simulink model "Inverter_pq_comp_sat_sim"  (R2023b)
settings: Solver=FixedStepDiscrete  StartTime=0.0  StopTime=2  RelTol=1e-3  EnableMultiTasking=on
InitFcn:
  | %% Definition of the parameters
  | 
  | Parameter_Definition
  | 
  | %% Damping
  | 
  | Rd = 3.9;
  | 
  | %% PRes Gains Calculation
  | 
  | % Definicao das grandezas
  | w_cl = 1j*2*pi*1200;  % Phase Crossing Frequency
  | no   = 1;           % Integral Resonant Constant
  | A    = 1;             % Carrier Amplitude
  | 
  | % Kp calculation
  | a0 = 1;
  | a1 = Rd*Cf;
  | b0 = 0;
  | b1 = Lf+Lg;
  | b2 = Rd*Lf*Cf+Rd*Lg*Cf;
  | b3 = Lf*Lg*Cf;
  | 
  | G_lcl = (a1*w_cl+a0)/(b3*w_cl^3+b2*w_cl^2+b1*w_cl+b0);
  | % G_lcl = 1/((Lf+Lg)*w_cl+Rf);
  | 
  | G_PWM = (1/A)*(1-w_cl*Ts/4)/(1+w_cl*Ts/4);
  | 
  | G_wc  = (Vdc/2)*(1/I_base)*G_lcl*G_PWM;
  | 
  | G_wc_abs = abs(G_wc);
  | 
  | Kp = 1/G_wc_abs;
  | 
  | % Discretized Controller Gains
  | ressonance_list = [1,5,7,11,13];
  | 
  | n_res = length(ressonance_list);
  | a = zeros(2,n_res);
  | b = zeros(2,n_res);
  | Ki_res = zeros(1,n_res);
  | 
  | % for i = 1:n_res
  | %   k = ressonance_list(i);
  | %   Ki_res(i) = (2.2*Kp)/(no*T_gr);
  | %   a(i) = (2*Ki_res(i)*Ts)/(4+((k*w_gr)^2)*Ts^2);
  | %   b(i) = (-8+2*((k*w_gr)^2)*Ts^2)/(4+((k*w_gr)^2)*Ts^2);
  | % end
  | 
  | % wc is the cutoff frequency/damping factor in rad/s
  | wc = 2;
  | 
  | for i = 1:n_res
  |   k = ressonance_list(i);
  |   wk = k * w_gr; % Resonant frequency for this harmonic
  | 
  |   Ki_res(i) = (2.2*Kp)/(0.8*no*T_gr);
  | 
  |   % 1. Calculate the common denominator
  |   den = 4 + 4*wc*Ts + (wk^2)*(Ts^2);
  | ... (+14 lines)
values from neighbouring files (symbols this model uses):
  a1_sogi = single(2*(w0_sogi^2-c_sogi^2)/den0_sogi)    [Parameter_Definition.m]
  a2_sogi = single((c_sogi^2                 - k_sogi*w0_sogi*c_sogi                 + w0_sogi^2)/den0_sogi)    [Parameter_Definition.m]
  bD_sogi = single(k_sogi*w0_sogi*c_sogi/den0_sogi)    [Parameter_Definition.m]
  bQ_sogi = single(k_sogi*w0_sogi^2/den0_sogi)    [Parameter_Definition.m]
  Cdc = 1.5e-3    (= 0.0015)    [Parameter_Definition.m]
  Cf = 5e-6    (= 5e-06)    [Parameter_Definition.m]
  f_gr = 60    [Parameter_Definition.m]
  I_base = S_base/(sqrt(3)*V_gr)    [Parameter_Definition.m]
  Lf = 1e-3    (= 0.001)    [Parameter_Definition.m]
  Lg = 0.5e-3    (= 0.0005)    [Parameter_Definition.m]
  Rdc = 0.1/(2*pi*60*Cdc)    (= 0.176838825658)    [Parameter_Definition.m]
  Rf = 0.1*Xf    (= 0.0376991118431)    [Parameter_Definition.m]
  Rg = 0.1*Xg    (= 0.0188495559215)    [Parameter_Definition.m]
  S_base = S_rated    (= 1000)    [Parameter_Definition.m]
  Ts = 2*(4167)/100e6    (= 8.334e-05)    [Parameter_Definition.m]
  Tstep = Ts/1000    (= 8.334e-08)    [Parameter_Definition.m]
  V_base = sqrt(3)*V_gr    [Parameter_Definition.m]
  V_gr = 127    [Parameter_Definition.m]
  Vdc = 800    [Parameter_Definition.m]
  Vdc_base = Vdc    (= 800)    [Parameter_Definition.m]
  w_gr = 2*pi*f_gr    (= 376.991118431)    [Parameter_Definition.m]
undefined symbols (not defined in the file or in its folder): gH_LUT, gQ_LUT, gV_LUT, lH_vetor, lQ_vetor, lV_vetor
libraries: spsSeriesRLCBranchLib x22, spsIGBTDiodeLib x12, spsCurrentMeasurementLib x9, spsVoltageMeasurementLib x5, c2837xDlib x4, spsACVoltageSourceLib x3, spsGroundLib x3, spsDCVoltageSourceLib x2, spsTriangleGeneratorLib x1, simulink x1, eeRmsMeasurement x1, spsTHDLib x1
(part 2 of 3)

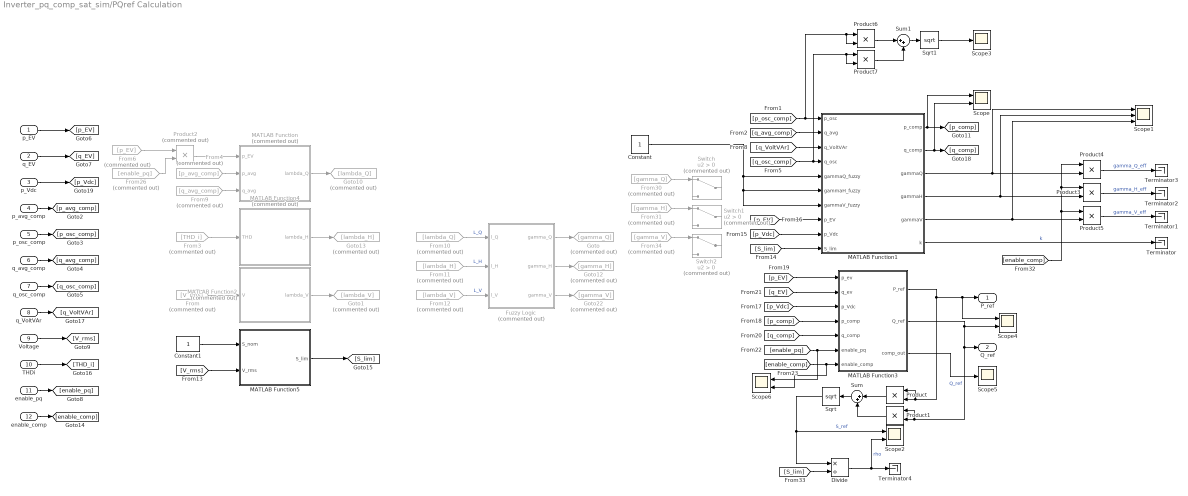
== system Inverter_pq_comp_sat_sim/PQref Calculation ==
  p_EV : Inport
  q_EV : Inport  Port=2
  p_Vdc : Inport  Port=3
  p_avg_comp : Inport  Port=4
  p_osc_comp : Inport  Port=5
  q_avg_comp : Inport  Port=6
  q_osc_comp : Inport  Port=7
  q_VoltVAr : Inport  Port=8
  Voltage : Inport  Port=9
  THDi : Inport  Port=10
  enable_pq : Inport  Port=11
  enable_comp : Inport  Port=12
  Constant : Constant  OutDataTypeStr=single  SampleTime=Ts
  Constant1 : Constant  OutDataTypeStr=single
  Divide : Product  Inputs=*/
  From : From  Commented=on  GotoTag=V_rms
  From10 : From  Commented=on  GotoTag=lambda_Q
  From11 : From  Commented=on  GotoTag=lambda_H
  From12 : From  Commented=on  GotoTag=lambda_V
  From26 : From  Commented=on  GotoTag=enable_pq
  From3 : From  Commented=on  GotoTag=THD_i
  From30 : From  Commented=on  GotoTag=gamma_Q
  From31 : From  Commented=on  GotoTag=gamma_H
  From34 : From  Commented=on  GotoTag=gamma_V
  From4 : From  Commented=on  GotoTag=p_avg_comp
  From6 : From  Commented=on  GotoTag=p_EV
  From9 : From  Commented=on  GotoTag=q_avg_comp
  Fuzzy Logic : Subsystem  Commented=on
  Goto : Goto  Commented=on  GotoTag=gamma_Q
  Goto1 : Goto  Commented=on  GotoTag=lambda_V
  Goto10 : Goto  Commented=on  GotoTag=lambda_Q
  Goto12 : Goto  Commented=on  GotoTag=gamma_H
  Goto13 : Goto  Commented=on  GotoTag=lambda_H
  Goto22 : Goto  Commented=on  GotoTag=gamma_V
  MATLAB Function : MATLAB Function  Commented=on  TreatAsAtomicUnit=on
  MATLAB Function1 : MATLAB Function  TreatAsAtomicUnit=on
  MATLAB Function2 : MATLAB Function  Commented=on  TreatAsAtomicUnit=on
  MATLAB Function3 : MATLAB Function  TreatAsAtomicUnit=on
  MATLAB Function4 : MATLAB Function  Commented=on  TreatAsAtomicUnit=on
  MATLAB Function5 : MATLAB Function  TreatAsAtomicUnit=on
  Product{,1,3..7} (7 alike) : Product
  Product2 : Product  Commented=on
  Scope{,2,4,6} (4 alike) : Scope  NumInputPorts=2
  Scope1 : Scope  NumInputPorts=3
  Scope3 : Scope
  Scope5 : Scope
  Sqrt : Sqrt
  Sqrt1 : Sqrt
  Sum : Sum  Inputs=|++
  Sum1 : Sum  Inputs=|++
  Switch : Switch  Commented=on  Criteria=u2 > Threshold  SaturateOnIntegerOverflow=off  InputSameDT=off
  Switch1 : Switch  Commented=on  Criteria=u2 > Threshold  SaturateOnIntegerOverflow=off  InputSameDT=off
  Switch2 : Switch  Commented=on  Criteria=u2 > Threshold  SaturateOnIntegerOverflow=off  InputSameDT=off
  Terminator{,1..4} (5 alike) : Terminator
  P_ref : Outport
  Q_ref : Outport  Port=2
  wires:
  Product3/1 -> Terminator2/1  "gamma_H_eff"
  From34/1 -> Switch2/1
  MATLAB Function3/1(P_ref) -> Product/2, Product/1, Scope4/1, P_ref/1
  [q_EV] -> MATLAB Function3/2(q_ev)
  Divide/1 -> Scope2/2, Terminator4/1  "rho"
  From31/1 -> Switch1/1
  Product2/1 -> MATLAB Function/1(p_EV)
  MATLAB Function1/6(k) -> Terminator/1  "k"
  Fuzzy Logic/3(gamma_V) -> Goto22/1
  Product/1 -> Sum/1
  MATLAB Function3/2(Q_ref) -> Product1/1, Product1/2, Q_ref/1, Scope4/2  "Q_ref"
  MATLAB Function1/5(gammaV) -> Scope1/3, Product5/2
  MATLAB Function1/4(gammaH) -> Scope1/2, Product3/2
  Sum/1 -> Sqrt/1
  Product5/1 -> Terminator1/1  "gamma_V_eff"
  MATLAB Function5/1(S_lim) -> [S_lim]
  [S_lim] -> Divide/2
  [enable_comp] -> Product4/1, Product3/1, Product5/1
  From9/1 -> MATLAB Function/3(q_avg)
  p_EV/1 -> [p_EV]
  p_osc_comp/1 -> [p_osc_comp]
  p_Vdc/1 -> [p_Vdc]
  Sqrt/1 -> Divide/1, Scope2/1  "S_ref"
  Constant1/1 -> MATLAB Function5/1(S_nom)
  From12/1 -> Fuzzy Logic/3(l_V)  "L_V"
  [V_rms] -> MATLAB Function5/2(V_rms)
  From10/1 -> Fuzzy Logic/1(l_Q)  "L_Q"
  [p_EV] -> MATLAB Function1/8(p_EV)
  Fuzzy Logic/2(gamma_H) -> Goto12/1
  From11/1 -> Fuzzy Logic/2(l_H)  "L_H"
  MATLAB Function1/2(q_comp) -> Scope/2, [q_comp]
  [p_osc_comp] -> MATLAB Function1/1(p_osc), Product6/2, Product6/1
  Product1/1 -> Sum/2
  [q_osc_comp] -> Product7/2, Product7/1, MATLAB Function1/4(q_osc)
  MATLAB Function1/3(gammaQ) -> Scope1/1, Product4/2
  [p_Vdc] -> MATLAB Function3/3(p_Vdc)
  Fuzzy Logic/1(gamma_Q) -> Goto/1
  q_EV/1 -> [q_EV]
  [p_Vdc] -> MATLAB Function1/9(p_Vdc)
  MATLAB Function1/1(p_comp) -> Scope/1, [p_comp]
  [S_lim] -> MATLAB Function1/10(S_lim)
  [q_VoltVAr] -> MATLAB Function1/3(q_VoltVAr)
  [p_EV] -> MATLAB Function3/1(p_ev)
  [q_comp] -> MATLAB Function3/5(q_comp)
  q_avg_comp/1 -> [q_avg_comp]
  enable_comp/1 -> [enable_comp]
  [enable_pq] -> Scope6/1, MATLAB Function3/6(enable_pq)
  From/1 -> MATLAB Function2/1(V)
  enable_pq/1 -> [enable_pq]
  MATLAB Function/1(lambda_Q) -> Goto10/1
  MATLAB Function4/1(lambda_H) -> Goto13/1
  THDi/1 -> [THD_i]
  [enable_comp] -> Scope6/2, MATLAB Function3/7(enable_comp)
  From3/1 -> MATLAB Function4/1(THD)
  [p_comp] -> MATLAB Function3/4(p_comp)
  MATLAB Function2/1(lambda_V) -> Goto1/1
  q_osc_comp/1 -> [q_osc_comp]
  Voltage/1 -> [V_rms]
  p_avg_comp/1 -> [p_avg_comp]
  q_VoltVAr/1 -> [q_VoltVAr]
  From6/1 -> Product2/1
  From4/1 -> MATLAB Function/2(p_avg)
  From30/1 -> Switch/1
  [q_avg_comp] -> MATLAB Function1/2(q_avg)
  Product4/1 -> Terminator3/1  "gamma_Q_eff"
  From26/1 -> Product2/2
  Constant/1 -> MATLAB Function1/7(gammaV_fuzzy), MATLAB Function1/6(gammaH_fuzzy), MATLAB Function1/5(gammaQ_fuzzy)
  Sum1/1 -> Sqrt1/1
  Product7/1 -> Sum1/2
  Product6/1 -> Sum1/1
  Sqrt1/1 -> Scope3/1
  MATLAB Function3/3(comp_out) -> Scope5/1

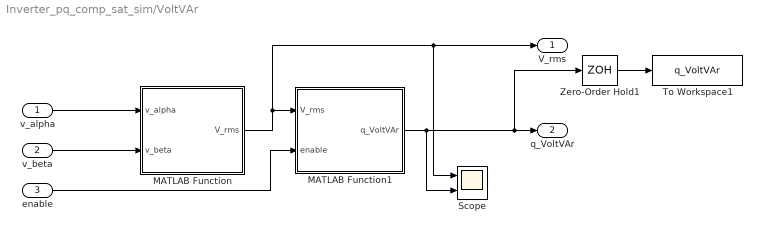
== system Inverter_pq_comp_sat_sim/VoltVAr ==
  v_alpha : Inport
  v_beta : Inport  Port=2
  enable : Inport  Port=3
  MATLAB Function : MATLAB Function  TreatAsAtomicUnit=on
  MATLAB Function1 : MATLAB Function  TreatAsAtomicUnit=on
  Scope : Scope  NumInputPorts=2
  To Workspace1 : ToWorkspace  VariableName=q_VoltVAr  SaveFormat=Timeseries  SampleTime=-1
  Zero-Order Hold1 : ZeroOrderHold  SampleTime=Ts
  V_rms : Outport
  q_VoltVAr : Outport  Port=2
  wires:
  MATLAB Function1/1(q_VoltVAr) -> Zero-Order Hold1/1, q_VoltVAr/1, Scope/2
  MATLAB Function/1(V_rms) -> Scope/1, V_rms/1, MATLAB Function1/1(V_rms)
  v_alpha/1 -> MATLAB Function/1(v_alpha)
  v_beta/1 -> MATLAB Function/2(v_beta)
  enable/1 -> MATLAB Function1/2(enable)
  Zero-Order Hold1/1 -> To Workspace1/1

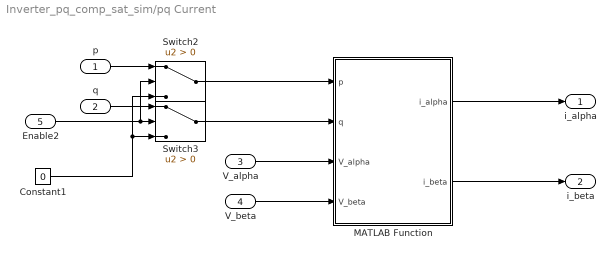
== system Inverter_pq_comp_sat_sim/pq Current ==
  p : Inport
  q : Inport  Port=2
  V_alpha : Inport  Port=3
  V_beta : Inport  Port=4
  Enable2 : Inport  Port=5
  Constant1 : Constant  Value=0
  MATLAB Function : MATLAB Function  TreatAsAtomicUnit=on
  Switch2 : Switch  Criteria=u2 > Threshold  SaturateOnIntegerOverflow=off  InputSameDT=off
  Switch3 : Switch  Criteria=u2 > Threshold  SaturateOnIntegerOverflow=off  InputSameDT=off
  i_alpha : Outport
  i_beta : Outport  Port=2
  wires:
  V_beta/1 -> MATLAB Function/4(V_beta)
  V_alpha/1 -> MATLAB Function/3(V_alpha)
  MATLAB Function/1(i_alpha) -> i_alpha/1
  MATLAB Function/2(i_beta) -> i_beta/1
  p/1 -> Switch2/1
  Switch3/1 -> MATLAB Function/2(q)
  q/1 -> Switch3/1
  Constant1/1 -> Switch2/3, Switch3/3
  Enable2/1 -> Switch2/2, Switch3/2
  Switch2/1 -> MATLAB Function/1(p)

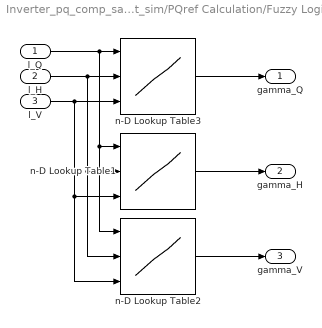
== system Inverter_pq_comp_sat_sim/PQref Calculation/Fuzzy Logic ==
  l_Q : Inport
  l_H : Inport  Port=2
  l_V : Inport  Port=3
  n-D Lookup Table1 : Lookup_n-D  NumberOfTableDimensions=3  BreakpointsForDimension1=lQ_vetor  BreakpointsForDimension2=lH_vetor  BreakpointsForDimension3=lV_vetor  Table=gH_LUT  InternalRulePriority=Speed  RndMeth=Simplest
      settings: InputPortMap=u0,u1,u2
  n-D Lookup Table2 : Lookup_n-D  NumberOfTableDimensions=3  BreakpointsForDimension1=lQ_vetor  BreakpointsForDimension2=lH_vetor  BreakpointsForDimension3=lV_vetor  Table=gV_LUT  InternalRulePriority=Speed  RndMeth=Simplest
      settings: InputPortMap=u0,u1,u2
  n-D Lookup Table3 : Lookup_n-D  NumberOfTableDimensions=3  BreakpointsForDimension1=lQ_vetor  BreakpointsForDimension2=lH_vetor  BreakpointsForDimension3=lV_vetor  Table=gQ_LUT  InternalRulePriority=Speed  RndMeth=Simplest
      settings: InputPortMap=u0,u1,u2
  gamma_Q : Outport
  gamma_H : Outport  Port=2
  gamma_V : Outport  Port=3
  wires:
  l_V/1 -> n-D Lookup Table3/3, n-D Lookup Table2/3, n-D Lookup Table1/3
  l_Q/1 -> n-D Lookup Table3/1, n-D Lookup Table2/1, n-D Lookup Table1/1
  l_H/1 -> n-D Lookup Table3/2, n-D Lookup Table2/2, n-D Lookup Table1/2
  n-D Lookup Table3/1 -> gamma_Q/1
  n-D Lookup Table1/1 -> gamma_H/1
  n-D Lookup Table2/1 -> gamma_V/1

== matlab function Inverter_pq_comp_sat_sim/RMS_fcn4 ==
  data: RMSin input; yout output
function yout = fcn(RMSin)

win = 200;

persistent sampleRMS
    if isempty(sampleRMS)
        sampleRMS = single(0.0);
    end
    if sampleRMS>=win
        sampleRMS = single(0.0);
    end

persistent RMSout
if isempty(RMSout)
    RMSout = single(0.0);
end    
persistent sumRMS
if isempty(sumRMS)
    sumRMS = single(0.0);
end
persistent RMSinArray
     if isempty(RMSinArray)
         RMSinArray = zeros(1,win);
     end

sampleRMS = sampleRMS + 1;      

%RMS of Input Signal
sumRMS = sumRMS + RMSin*RMSin - RMSinArray(1,sampleRMS);
RMSinArray(1,sampleRMS) = RMSin*RMSin;
if sumRMS>=0.0
    RMSout = sqrt(sumRMS/win);
end

%RMSout = RMSout_temp;

yout = RMSout;

== matlab function Inverter_pq_comp_sat_sim/RMS_fcn5 ==
  data: RMSin input; yout output
function yout = fcn(RMSin)

win = 200;

persistent sampleRMS
    if isempty(sampleRMS)
        sampleRMS = single(0.0);
    end
    if sampleRMS>=win
        sampleRMS = single(0.0);
    end

persistent RMSout
if isempty(RMSout)
    RMSout = single(0.0);
end    
persistent sumRMS
if isempty(sumRMS)
    sumRMS = single(0.0);
end
persistent RMSinArray
     if isempty(RMSinArray)
         RMSinArray = zeros(1,win);
     end

sampleRMS = sampleRMS + 1;      

%RMS of Input Signal
sumRMS = sumRMS + RMSin*RMSin - RMSinArray(1,sampleRMS);
RMSinArray(1,sampleRMS) = RMSin*RMSin;
if sumRMS>=0.0
    RMSout = sqrt(sumRMS/win);
end

%RMSout = RMSout_temp;

yout = RMSout;

== matlab function Inverter_pq_comp_sat_sim/Compensation Reference/MATLAB Function1 ==
  data: i_alpha input; p_avg output; i_beta input; v_alpha input; v_beta input; p_osc output; q_avg output; q_osc output
function [p_avg, p_osc, q_avg, q_osc] = pqCalc(i_alpha, i_beta, v_alpha, v_beta)
    % Initial logic and parameters are validated. 
    % Standard processing applied for spatial vector alignment.

    persistent buffer_p buffer_q sum_p sum_q idx
    window = 200; % Must match your 12000Hz/60Hz window size exactly
    
    if isempty(buffer_p)
        buffer_p = zeros(window, 1);
        buffer_q = zeros(window, 1);
        sum_p = single(0.0);
        sum_q = single(0.0);
        idx = 1;
    end
    
    % Final transformation: Strip scaling coefficients to match I_total_sq domain
    p = (v_alpha * i_alpha) + (v_beta * i_beta);
    q = (v_beta * i_alpha) - (v_alpha * i_beta);
    
    % Align filter topology to match current/voltage sliding window
    old_p = buffer_p(idx);
    old_q = buffer_q(idx);
    
    buffer_p(idx) = p;
    buffer_q(idx) = q;
    
    sum_p = sum_p + p - old_p;
    sum_q = sum_q + q - old_q;
    
    idx = idx + 1;
    if idx > window
        idx = 1;
    end
    
    p_avg = sum_p / window;
    q_avg = sum_q / window;
    
    p_osc = p - p_avg;
    q_osc = q - q_avg;
end

== matlab function Inverter_pq_comp_sat_sim/MATLAB Function11 ==
  data: i_rms input; error_overcurrent output; error_ac_overvoltage output; error_dc_overvoltage output; error_unbalance output; error_low_Vdc output; enable_contactor_out output; enable_PreCharge_out output; enable_PWM_out output; enable_PQ_out output; enable_comp_out output; enable_Feedforward_out output; I_limit input; V_rms input; V_limit input; V_dc input; Vdc_limit input; V_unb input; Vunb_limit input; enable_relay input; enable_PWM input; enable_PreCharge input; enable_PQ input; enable_comp input; error_reset input; error_reset_out output; out_gpio output
function [error_overcurrent, error_ac_overvoltage, error_dc_overvoltage, error_unbalance, error_low_Vdc, enable_contactor_out, enable_PreCharge_out, enable_PWM_out, enable_PQ_out, enable_comp_out, enable_Feedforward_out, error_reset_out, out_gpio] = TNPC_Protection(i_rms, I_limit, V_rms, V_limit, V_dc, Vdc_limit, V_unb, Vunb_limit, enable_relay, enable_PWM, enable_PreCharge, enable_PQ, enable_comp, error_reset)

% Persistent variables definition
persistent error_flag
persistent error_overcurrent_p
persistent error_ac_overvoltage_p
persistent error_dc_overvoltage_p
persistent error_unbalance_p
persistent error_low_Vdc_p
persistent count_I_limit
if isempty(error_flag)
    error_flag = single(0);
    error_overcurrent_p    = single(0);
    error_ac_overvoltage_p = single(0);
    error_dc_overvoltage_p = single(0);
    error_unbalance_p      = single(0);
    error_low_Vdc_p        = single(0);
    count_I_limit          = int16(0);
end


out_Feedforward = single(0.0);
% Count to keep high current limit in first 15 cycles
if enable_relay == 1
    if count_I_limit < 10*200
        I_limit = single(100.0);
        count_I_limit = count_I_limit + 1;
        out_Feedforward = single(1.0);
    elseif count_I_limit < 15*200
        I_limit = single(100.0);
        count_I_limit = count_I_limit + 1;
        out_Feedforward = single(0.0);
    end
end

enable_Feedforward_out = out_Feedforward;

% Check for errors
if max(i_rms) > I_limit
    error_overcurrent = single(1);
    error_overcurrent_p = single(1);
else
    error_overcurrent = single(0);
end

if V_dc > Vdc_limit
    error_dc_overvoltage = single(1);
    error_dc_overvoltage_p = single(1);
else
    error_dc_overvoltage = single(0);  
end

if V_unb > Vunb_limit
    error_unbalance = single(1);
    error_unbalance_p = single(1);
else
    error_unbalance = single(0);
end

if max(V_rms) > V_limit
    error_ac_overvoltage = single(1);
    error_ac_overvoltage_p = single(1);
else
    error_ac_overvoltage = single(0);  
end

if V_dc*500 < sqrt(2)*max(V_rms)*250
    error_low_Vdc = single(1);
    error_low_Vdc_p = single(1);
else
    error_low_Vdc = single(0);
end

% Raise the error flag
if (error_overcurrent == 1) || (error_dc_overvoltage == 1) || (error_unbalance == 1) || (error_ac_overvoltage == 1) || (error_low_Vdc == 1)
    error_flag = single(1);
end

% Reset logic
if error_flag == 1 && error_reset == 1 && error_overcurrent == 0 && error_dc_overvoltage == 0 && error_ac_overvoltage == 0 && error_unbalance == 0 && error_low_Vdc == 0
    % Clear the persistent variables
    error_flag = single(0);
    error_overcurrent_p    = single(0);
    error_ac_overvoltage_p = single(0);
    error_dc_overvoltage_p = single(0);
    error_unbalance_p      = single(0);
    error_low_Vdc_p        = single(0);
    count_I_limit          = int16(0);
    % Send 0 to the reset signal
    error_reset_out = single(0);
else
    error_reset_out = error_reset;
end

% Enable signals output
if error_flag == 1
    enable_contactor_out = single(0);
    enable_PWM_out       = single(0);
    enable_PreCharge_out = single(0);
    enable_PQ_out        = single(0);
    enable_comp_out      = single(0);
else
    enable_contactor_out = enable_relay;
    enable_PWM_out       = enable_PWM;
    enable_PreCharge_out = enable_PreCharge;
    enable_PQ_out        = enable_PQ;
    enable_comp_out      = enable_comp;
end

if (error_overcurrent_p == 1) || (error_dc_overvoltage_p == 1) || (error_unbalance_p == 1) || (error_ac_overvoltage_p == 1) || (error_low_Vdc_p == 1)
    out_gpio = single(1);
else
    out_gpio = single(0);
end

== matlab function Inverter_pq_comp_sat_sim/PQref Calculation/MATLAB Function ==
  data: p_EV input; p_avg input; lambda_Q output; q_avg input
function lambda_Q  = lambda_Q_calc(p_EV, p_avg, q_avg)

lQ_min = sqrt(1-0.75^2);

lQ = q_avg/sqrt((-p_EV + p_avg)^2+q_avg^2);
lambda_Q = lQ/lQ_min;
lambda_Q = max(-1,min(1,lambda_Q));

== matlab function Inverter_pq_comp_sat_sim/Current Controller/RMS_fcn ==
  data: RMSin input; yout output
function yout = fcn(RMSin)

win = 200;

persistent sampleRMS
    if isempty(sampleRMS)
        sampleRMS = single(0.0);
    end
    if sampleRMS>=win
        sampleRMS = single(0.0);
    end

persistent RMSout
if isempty(RMSout)
    RMSout = single(0.0);
end    
persistent sumRMS
if isempty(sumRMS)
    sumRMS = single(0.0);
end
persistent RMSinArray
     if isempty(RMSinArray)
         RMSinArray = zeros(1,win);
     end

sampleRMS = sampleRMS + 1;      

%RMS of Input Signal
sumRMS = sumRMS + RMSin*RMSin - RMSinArray(1,sampleRMS);
RMSinArray(1,sampleRMS) = RMSin*RMSin;
if sumRMS>=0.0
    RMSout = sqrt(sumRMS/win);
end

%RMSout = RMSout_temp;

yout = RMSout;

== matlab function Inverter_pq_comp_sat_sim/PQref Calculation/MATLAB Function1 ==
  data: p_osc input; q_avg input; q_VoltVAr input; q_osc input; gammaQ_fuzzy input; gammaH_fuzzy input; gammaV_fuzzy input; p_comp output; q_comp output; p_EV input; p_Vdc input; S_lim input; gammaQ output; gammaH output; gammaV output; k output
function [p_comp, q_comp, gammaQ, gammaH, gammaV, k] = PQCompCalc( ...
    p_osc, q_avg, q_VoltVAr, q_osc, ...
    gammaQ_fuzzy, gammaH_fuzzy, gammaV_fuzzy, p_EV, p_Vdc, S_lim)
%#codegen

    window = 200;
    eps_power = single(1e-9);

    % Monotonic maximum deque for S_total
    persistent q_Stotal;
    persistent pos_Stotal;

    % Monotonic minimum deque for k
    persistent q_k;
    persistent pos_k;

    persistent t;

    if isempty(t)
        q_Stotal = zeros(window, 2, "single");
        q_k      = zeros(window, 2, "single");

        pos_Stotal = 0;
        pos_k = 0;
        t = 0;
    end

    % ---------------------------------------------------------------------
    % Sample counter
    % ---------------------------------------------------------------------
    t = t + 1;

    if t > 1000000
        for i = 1:pos_Stotal
            q_Stotal(i, 2) = q_Stotal(i, 2) - 1000000;
        end

        for i = 1:pos_k
            q_k(i, 2) = q_k(i, 2) - 1000000;
        end

        t = t - 1000000;
    end

    % Maintain your adopted p_Vdc sign convention.
    p_0 = p_EV - p_Vdc;

    % Ensure a nonnegative limit
    S_lim_safe = max(S_lim, single(0.0));

    % =====================================================================
    % 1. ROLLING MAXIMUM OF THE TOTAL REQUIRED POWER
    % =====================================================================
    S_tot_inst = sqrt( ...
        (p_0 + p_osc)^2 + ...
        (q_avg + q_VoltVAr + q_osc)^2);

    % ---------------------------------------------------------------------
    % IMPORTANT CORRECTION:
    % Remove expired samples BEFORE inserting the new sample.
    % ---------------------------------------------------------------------
    while (pos_Stotal > 0) && ...
          (q_Stotal(1, 2) <= t - window)

        for i = 1:(pos_Stotal - 1)
            q_Stotal(i, :) = q_Stotal(i + 1, :);
        end

        pos_Stotal = pos_Stotal - 1;
    end

    % Remove samples dominated by the current value
    while (pos_Stotal > 0) && ...
          (q_Stotal(pos_Stotal, 1) <= S_tot_inst)

        pos_Stotal = pos_Stotal - 1;
    end

    % Defensive protection. With the expiration order corrected,
    % this condition should normally never occur.
    if pos_Stotal >= window
        for i = 1:(window - 1)
            q_Stotal(i, :) = q_Stotal(i + 1, :);
        end

        pos_Stotal = window - 1;
    end

    % Insert current sample
    pos_Stotal = pos_Stotal + 1;
    q_Stotal(pos_Stotal, 1) = S_tot_inst;
    q_Stotal(pos_Stotal, 2) = t;

    % Maximum is always stored at the beginning of the deque
    S_total_max = q_Stotal(1, 1);

    % =====================================================================
    % 2. FUZZY-WEIGHTED COMPENSATION REFERENCES
    % =====================================================================
    p_fuz = gammaH_fuzzy * p_osc;

    q_fuz = gammaQ_fuzzy * q_avg + gammaV_fuzzy * q_VoltVAr + gammaH_fuzzy  * q_osc;

    % Maximum scaling allowed without overcompensation
    lambda_max = max(gammaV_fuzzy, max(gammaQ_fuzzy, gammaH_fuzzy));

    if lambda_max > eps_power
        k_cap = single(1.0) / lambda_max;
    else
        % Both fuzzy weights are zero. The value of k has no effect
        % because p_fuz = q_fuz = 0.
        k_cap = single(1.0);
    end

    % Quadratic coefficients
    a = p_fuz^2 + q_fuz^2;
    b = 2 * p_0 * p_fuz;
    c = p_0^2 - S_lim_safe^2;

    % Indicates whether a meaningful k value exists at this sample
    update_k_queue = true;

    if a < eps_power
        % No ancillary-service vector exists at this instant.
        %
        % Do not use k_inst = 0, because it would remain in the minimum
        % queue for one complete grid cycle and temporarily block
        % compensation when a load is connected.
        k_inst = k_cap;
        update_k_queue = false;

    else
        delta = b^2 - 4 * a * c;

        if delta < 0
            % A slightly negative value can be caused by rounding.
            % A significantly negative value normally indicates that
            % the requested operating point is infeasible.
            delta = single(0.0);
        end

        % Largest root: maximum positive scaling that satisfies S_lim
        k_inst = (-b + sqrt(delta)) / (2 * a);

        % Prevent negative scaling and overcompensation
        k_inst = max(k_inst, single(0.0));
        k_inst = min(k_inst, k_cap);
    end

    % =====================================================================
    % 3. ROLLING MINIMUM OF k
    % =====================================================================

    % Remove all expired k samples before inserting a new one
    while (pos_k > 0) && (q_k(1, 2) <= t - window)

        for i = 1:(pos_k - 1)
            q_k(i, :) = q_k(i + 1, :);
        end

        pos_k = pos_k - 1;
    end

    % Only store k when the compensation vector is meaningful
    if update_k_queue

        % Remove values dominated by the current minimum candidate
        while (pos_k > 0) && ...
              (q_k(pos_k, 1) >= k_inst)

            pos_k = pos_k - 1;
        end

        % Defensive overflow protection
        if pos_k >= window
            for i = 1:(window - 1)
                q_k(i, :) = q_k(i + 1, :);
            end

            pos_k = window - 1;
        end

        % Insert current k
        pos_k = pos_k + 1;
        q_k(pos_k, 1) = k_inst;
        q_k(pos_k, 2) = t;
    end

    % Obtain the rolling minimum
    if pos_k > 0
        k_min = q_k(1, 1);
    else
        % No valid compensation demand has been observed
        k_min = k_cap;
    end

    % Apply current-sample protection again because the fuzzy
    % weights, and therefore k_cap, may have changed.
    k_min = max(k_min, single(0.0));
    k_min = min(k_min, k_cap);

    % =====================================================================
    % 4. FINAL COMPENSATION REFERENCES
    % =====================================================================
    if S_total_max <= S_lim_safe

        % Full compensation is feasible
        p_comp = p_osc;
        q_comp = q_avg + q_VoltVAr + q_osc;

        gammaQ = single(1.0);
        gammaH = single(1.0);
        gammaV = single(1.0);
        k = single(1.0);

    else

        % Insufficient converter capacity
        p_comp = k_min * p_fuz;
        q_comp = k_min * q_fuz;

        gammaQ = min(gammaQ_fuzzy * k_min, 1);
        gammaH  = min(gammaH_fuzzy  * k_min, 1);
        gammaV  = min(gammaV_fuzzy  * k_min, 1);
        k = k_min;
    end
end

== matlab function Inverter_pq_comp_sat_sim/MATLAB Function6 ==
  data: i_alpha input; p_avg output; i_beta input; v_alpha input; v_beta input; p_osc output; q_avg output; q_osc output
function [p_avg, p_osc, q_avg, q_osc] = pqCalc(i_alpha, i_beta, v_alpha, v_beta)
    % Initial logic and parameters are validated. 
    % Standard processing applied for spatial vector alignment.

    persistent buffer_p buffer_q sum_p sum_q idx
    window = 200; % Must match your 12000Hz/60Hz window size exactly
    
    if isempty(buffer_p)
        buffer_p = zeros(window, 1, "single");
        buffer_q = zeros(window, 1, "single");
        sum_p = single(0.0);
        sum_q = single(0.0);
        idx = 1;
    end
    
    % Final transformation: Strip scaling coefficients to match I_total_sq domain
    p = (v_alpha * i_alpha) + (v_beta * i_beta);
    q = (v_beta * i_alpha) - (v_alpha * i_beta);
    
    % Align filter topology to match current/voltage sliding window
    old_p = buffer_p(idx);
    old_q = buffer_q(idx);
    
    buffer_p(idx) = p;
    buffer_q(idx) = q;
    
    sum_p = sum_p + p - old_p;
    sum_q = sum_q + q - old_q;
    
    idx = idx + 1;
    if idx > window
        idx = 1;
    end
    
    p_avg = sum_p / window;
    q_avg = sum_q / window;
    
    p_osc = p - p_avg;
    q_osc = q - q_avg;
end

== matlab function Inverter_pq_comp_sat_sim/Current Controller/MATLAB Function2 ==
  data: alpha input; a output; beta input; b output; c output; aux output
function [a, b, c, aux] = abc(alpha, beta)

a = sqrt(2/3)*alpha;
b = sqrt(2/3)*(-1*alpha/2 + sqrt(3)*beta/2);
c = sqrt(2/3)*(-1*alpha/2 - sqrt(3)*beta/2);

max_mod = max(abs([a, b, c]));

if max_mod > 1
    % scale = 1/max_mod;
    % 
    % a = a*scale;
    % b = b*scale;
    % c = c*scale;

    aux = single(1.0);
else
    aux = single(0.0);
end

== matlab function Inverter_pq_comp_sat_sim/PQref Calculation/MATLAB Function2 ==
  data: V input; lambda_V output
function lambda_V = lambda_V_calc(V)

delta_V = 0.15;
V_min = 1-delta_V;
V_max = 1+delta_V;

lambda_V = (V-V_min)/(V_max-V_min);
lambda_V = max(0,min(1,lambda_V));

== matlab function Inverter_pq_comp_sat_sim/MATLAB Function3 ==
  data: a input; alpha output; b input; c input; beta output
function [alpha, beta] = alpha_beta(a, b, c)

alpha = sqrt(2/3)*(a - b/2 - c/2);
beta  = sqrt(2/3)*(sqrt(3)*b/2 - sqrt(3)*c/2);

== matlab function Inverter_pq_comp_sat_sim/pq Current/MATLAB Function ==
  data: p input; i_alpha output; q input; i_beta output; V_alpha input; V_beta input
function [i_alpha, i_beta] = pq_to_i(p, q, V_alpha, V_beta)

i_alpha = (1/(V_alpha^2+V_beta^2))*(V_alpha*p + V_beta*q);
i_beta  = (1/(V_alpha^2+V_beta^2))*(V_beta*p - V_alpha*q);

== matlab function Inverter_pq_comp_sat_sim/PQref Calculation/MATLAB Function3 ==
  data: p_ev input; P_ref output; q_ev input; p_Vdc input; p_comp input; q_comp input; enable_pq input; enable_comp input; Q_ref output; comp_out output
function [P_ref, Q_ref,comp_out] = PQ_ref(p_ev, q_ev, p_Vdc, p_comp, q_comp, enable_pq, enable_comp)

comp_out = 0;
if enable_pq == 0
    P_ref = -1*p_Vdc;
    Q_ref = single(0.0);
else
    if enable_comp == 0
        P_ref = p_ev - p_Vdc;
        Q_ref = q_ev;
    else
        P_ref = p_ev - p_Vdc + p_comp;
        Q_ref = q_ev + q_comp;
        comp_out = 1;
    end
end

== matlab function Inverter_pq_comp_sat_sim/PQref Calculation/MATLAB Function4 ==
  data: THD input; lambda_H output
function lambda_H  = lambda_H_calc(THD)

THD_min = 0;
THD_max = 0.3;

% Number of samples in the MAF window
% Set this equal to approximately one grid cycle
N_MAF = 200;

% ---------------------------------------------------------
% Moving Average Filter
% ---------------------------------------------------------
persistent buffer idx count running_sum

if isempty(buffer)
    buffer = zeros(1, N_MAF);
    idx = 1;
    count = 0;
    running_sum = 0;
end

% Remove oldest value from running sum
running_sum = running_sum - buffer(idx);

% Store new value
buffer(idx) = THD;

% Add new value to running sum
running_sum = running_sum + THD;

% Number of valid samples during startup
if count < N_MAF
    count = count + 1;
end

% Calculate moving average
THD = running_sum / count;

% Advance circular-buffer index
idx = idx + 1;

if idx > N_MAF
    idx = 1;
end

lambda_H = (THD - THD_min)/(THD_max - THD_min);
% Saturation [0,1]
lambda_H = max(0, min(1, lambda_H));

== matlab function Inverter_pq_comp_sat_sim/Compensation Reference/MATLAB Function ==
  data: i_alpha input; THDi output; i_beta input; v_alpha input; v_beta input; p_EV input; p_avg input; q_avg input
function THDi = THD_calc( ...
    i_alpha, i_beta, ...
    v_alpha, v_beta, ...
    p_EV, p_avg, q_avg)
%#codegen

    window = 200;
    epsilon = 1e-9;

    persistent buffer_I_total;
    persistent buffer_V;
    persistent sum_I_total;
    persistent sum_V;
    persistent idx;
    persistent count;

    if isempty(idx)
        buffer_I_total = zeros(window,1);
        buffer_V = zeros(window,1);

        sum_I_total = single(0.0);
        sum_V = single(0.0);

        idx = 1;
        count = 0;
    end

    % Load-current magnitude squared
    I_total_inst_sq = i_alpha^2 + i_beta^2;

    % Fundamental PCC-voltage magnitude squared
    V_inst_sq = v_alpha^2 + v_beta^2;

    % Remove oldest samples
    old_I = buffer_I_total(idx);
    old_V = buffer_V(idx);

    % Insert newest samples
    buffer_I_total(idx) = I_total_inst_sq;
    buffer_V(idx) = V_inst_sq;

    % Update moving sums
    sum_I_total = ...
        sum_I_total + I_total_inst_sq - old_I;

    sum_V = ...
        sum_V + V_inst_sq - old_V;

    idx = idx + 1;

    if idx > window
        idx = 1;
    end

    if count < window
        count = count + 1;
    end

    % Do not calculate THD before one complete cycle
    if count < window
        THDi = single(0.0);
        return;
    end

    % Squared total load-current magnitude
    IL_total_sq = max(sum_I_total/window,single(0.0));

    % Squared fundamental voltage magnitude
    V1_sq = max(sum_V/window,epsilon);

    % Fundamental LOAD current
    IL_fund_sq = ...
        (p_avg^2 + q_avg^2)/V1_sq;

    % Harmonic LOAD current
    IH_load_sq = max( ...
        IL_total_sq - IL_fund_sq, ...
        single(0.0));

    % Fundamental grid current including EV charging
    %
    % Current convention:
    % p_EV is negative during charging.
    p_total_fund = p_avg - p_EV;

    IT_fund_sq = ...
        (p_total_fund^2 + q_avg^2)/V1_sq;

    % Equivalent pre-compensation grid THD
    if IT_fund_sq <= epsilon
        THDi = single(0.0);
    else
        THDi = sqrt(IH_load_sq/IT_fund_sq);
    end
end

== matlab function Inverter_pq_comp_sat_sim/VoltVAr/MATLAB Function ==
  data: v_alpha input; V_rms output; v_beta input
function V_rms = VrmsCalc(v_alpha, v_beta)
    % #codegen
    window = 200;
    
    
    persistent buffer;
    persistent idx;
    persistent sum_vsq;
    
    % Inicialização
    if isempty(idx)
        buffer = zeros(window, 1);
        idx = 1;
        sum_vsq = single(0.0);
    end
    
    % 1. Calcula o quadrado da magnitude instantânea (V_alpha^2 + V_beta^2)
    v_sq_inst = v_alpha^2 + v_beta^2;
    
    % 2. Média Móvel Rápida (Soma o novo, subtrai o mais antigo do buffer)
    sum_vsq = sum_vsq - buffer(idx) + v_sq_inst;
    
    % Atualiza a memória com o novo valor
    buffer(idx) = v_sq_inst;
    
    % Avança o ponteiro circular
    idx = idx + 1;
    if idx > window
        idx = 1;
    end
    
    % 3. Calcula a média e extrai a raiz para obter o RMS
    % Garante que a soma não seja negativa por erro de precisão flutuante (max)
    v_sq_medio = max(sum_vsq / window, 0);
    
    % Equação final: V_rms = V_pico / sqrt(2) = sqrt(V_sq_medio / 2)
    V_rms = sqrt(v_sq_medio);
    
end

== matlab function Inverter_pq_comp_sat_sim/VoltVAr/MATLAB Function1 ==
  data: V_rms input; q_VoltVAr output; enable input
function q_VoltVAr = VoltVAr(V_rms, enable)

% Curve Definition
V1 = 0.9;
V2 = 0.96;
V3 = 1.03;
V4 = 1.10;

% Max Q processing
Q_max = single(1.0);

if enable == 0
    q_VoltVAr = single(0.0);
else
    if V_rms < V1
        q_VoltVAr = Q_max;
    else
        if V_rms < V2
            q_VoltVAr = Q_max*(V2 - V_rms)/(V2 - V1);
        else
            if V_rms < V3
                q_VoltVAr = single(0.0);
            else
               if V_rms < V4
                   q_VoltVAr = single(-1.0)*Q_max*(V_rms - V3)/(V4 - V3);
               else
                   q_VoltVAr = single(-1.0)*Q_max;
               end
            end
        end
    end
end

== matlab function Inverter_pq_comp_sat_sim/MATLAB Function5 ==
  data: a input; alpha output; b input; c input; beta output
function [alpha, beta] = alpha_beta(a, b, c)

alpha = sqrt(2/3)*(a - b/2 - c/2);
beta  = sqrt(2/3)*(sqrt(3)*b/2 - sqrt(3)*c/2);

== matlab function Inverter_pq_comp_sat_sim/Current Controller/PRes ==
  data: Kp input; a input; b input; errora input; ma output; errorb input; mb output; enable input
function [ma, mb] = PResCurrent(Kp, a, b, errora, errorb, enable)

%Controller modeled in abc frame, considering p.u. values

%%% Variables Definition
%%%%#########################################################
%%%%######################################################### 

nRes = length(a);

max_pu = single(1.0);

%Proportional part variable
%Phase a
persistent pia
    if isempty(pia)
        pia = single(0.0);
    end
%Phase b    
persistent pib
    if isempty(pib)
        pib = single(0.0);
    end 
    
%Resonant parts variables
%Phase a
persistent presa
    if isempty(presa)
        presa = zeros(1,nRes);
    end
persistent presa_1d %1 sample delay
    if isempty(presa_1d)
        presa_1d = zeros(1,nRes);
    end    
persistent presa_2d %2 samples delay
    if isempty(presa_2d)
        presa_2d = zeros(1,nRes);
    end
persistent presOUT_ia
    if isempty(presOUT_ia)
        presOUT_ia = single(0.0);
    end
    
%Phase b
persistent presb
    if isempty(presb)
        presb = zeros(1,nRes);
    end
persistent presb_1d %1 sample delay
    if isempty(presb_1d)
        presb_1d = zeros(1,nRes);
    end    
persistent presb_2d %2 samples delay
    if isempty(presb_2d)
        presb_2d = zeros(1,nRes);
    end
persistent presOUT_ib
    if isempty(presOUT_ib)
        presOUT_ib = single(0.0);
    end

%Error variables
%Phase a
% persistent errora %Actual error
%     if isempty(errora)
%         errora = 0.0;
%     end
persistent errora_0d %Actual error to delay
    if isempty(errora_0d)
        errora_0d = single(0.0);
    end
persistent errora_1d %1 sample delay
    if isempty(errora_1d)
        errora_1d = single(0.0);
    end    
persistent errora_2d %2 sample delay
    if isempty(errora_2d)
        errora_2d = single(0.0);
    end   
%Phase b
% persistent errorb %Actual error
%     if isempty(errorb)
%         errorb = 0.0;
%     end
persistent errorb_0d %Actual error to delay
    if isempty(errorb_0d)
        errorb_0d = single(0.0);
    end
persistent errorb_1d %1 sample delay
    if isempty(errorb_1d)
        errorb_1d = single(0.0);
    end    
persistent errorb_2d %2 sample delay
    if isempty(errorb_2d)
        errorb_2d = single(0.0);
    end

%%% Enable logic
%%%%#########################################################
%%%%#########################################################

if ~enable 
    % Define safe outputs
    ma = single(0.0);
    mb = single(0.0);
    mc = single(0.0);
    
    % Reset history registers for bumpless transfer
    pia = single(0.0); pib = single(0.0);
    
    presa       = zeros(1,nRes);
    presa_1d    = zeros(1,nRes);
    presa_2d    = zeros(1,nRes);
    presOUT_ia  = single(0.0);
    
    presb       = zeros(1,nRes);
    presb_1d    = zeros(1,nRes);
    presb_2d    = zeros(1,nRes);
    presOUT_ib  = single(0.0);
    
    errora_0d = single(0.0); errora_1d = single(0.0); errora_2d = single(0.0);
    errorb_0d = single(0.0); errorb_1d = single(0.0); errorb_2d = single(0.0);
    
    % Exit the function completely
    return; 
end

%%% PRes Current Controllers
%%%%#########################################################
%%%%#########################################################

%Proportional part
pia = errora*Kp;
pib = errorb*Kp;
    
    %Saturation - a
    if pia > max_pu 
        pia = max_pu;
    end
    if pia < -1*max_pu
        pia = -1*max_pu;
    end
    %Saturation - b
    if pib > max_pu
        pib = max_pu;
    end
    if pib < -1*max_pu
        pib = -1*max_pu;
    end   
    
    % %Anti-windup - a
    % if pia > 0.0
    %     limit_ia = max_pu - pia;
    % else
    %     limit_ia = 1 + pia;
    % end
    %  %Anti-windup - b
    % if pib > 0.0
    %     limit_ib = max_pu - pib;
    % else
    %     limit_ib = 1 + pib;
    % end
%     %Anti-windup - c
%     if pic > 0.0
%         limit_ic = max_pu - pic;
%     else
%         limit_ic = 1 + pic;
%     end    
    
    
%Resonant part
errora_2d = errora_1d;
errora_1d = errora_0d;
errora_0d = errora;

errorb_2d = errorb_1d;
errorb_1d = errorb_0d;
errorb_0d = errorb;
        
for i=1:nRes

    %leg a
    presa_2d(i) = presa_1d(i);
	presa_1d(i) = presa(i);
	presa(i) = a(1,i)*errora + a(2,i)*errora_2d - b(1,i)*presa_1d(i) - b(2,i)*presa_2d(i);    
    % if presa(i) > limit_ia
    %     presa(i) = limit_ia;
    % end
    % if presa(i) < -1*limit_ia
    %     presa(i) = -1*limit_ia;
    % end
 
    %leg b
    presb_2d(i) = presb_1d(i);
	presb_1d(i) = presb(i);
	presb(i) = a(1,i)*errorb + a(2,i)*errorb_2d - b(1,i)*presb_1d(i) - b(2,i)*presb_2d(i);    
    % if presb(i) > limit_ib
    %     presb(i) = limit_ib;
    % end
    % if presb(i) < -1*limit_ib
    %     presb(i) = -1*limit_ib;
    % end  
    
end

presOUT_ia = pia;
presOUT_ib = pib;

for i=1:nRes
    presOUT_ia = presOUT_ia + presa(i);
    presOUT_ib = presOUT_ib + presb(i);  
end

%Output for PWM
ma = presOUT_ia;
        % %Saturation - ta
        % if ma > max_pu 
        %     ma = max_pu;
        % end
        % if ma < -1*max_pu
        %     ma = -1*max_pu;
        % end

mb = presOUT_ib;
        % %Saturation - tb
        % if mb > max_pu 
        %     mb = max_pu;
        % end
        % if mb < -1*max_pu
        %     mb = -1*max_pu;
        % end
        
end

== matlab function Inverter_pq_comp_sat_sim/PQref Calculation/MATLAB Function5 ==
  data: S_nom input; S_lim output; V_rms input
function S_lim = S_lim_calc(S_nom, V_rms)

S_lim = min(S_nom, S_nom*V_rms);

== matlab function Inverter_pq_comp_sat_sim/MATLAB Function1 ==
  data: a input; alpha output; b input; c input; beta output
function [alpha, beta] = alpha_beta(a, b, c)

alpha = sqrt(2/3)*(a - b/2 - c/2);
beta  = sqrt(2/3)*(sqrt(3)*b/2 - sqrt(3)*c/2);

== matlab function Inverter_pq_comp_sat_sim/MATLAB Function7 ==
  data: i_alpha input; p_avg output; i_beta input; v_alpha input; v_beta input; p_osc output; q_avg output; q_osc output
function [p_avg, p_osc, q_avg, q_osc] = pqCalc(i_alpha, i_beta, v_alpha, v_beta)
    % Initial logic and parameters are validated. 
    % Standard processing applied for spatial vector alignment.

    persistent buffer_p buffer_q sum_p sum_q idx
    window = 200; % Must match your 12000Hz/60Hz window size exactly
    
    if isempty(buffer_p)
        buffer_p = zeros(window, 1, "single");
        buffer_q = zeros(window, 1, "single");
        sum_p = single(0.0);
        sum_q = single(0.0);
        idx = 1;
    end
    
    % Final transformation: Strip scaling coefficients to match I_total_sq domain
    p = (v_alpha * i_alpha) + (v_beta * i_beta);
    q = (v_beta * i_alpha) - (v_alpha * i_beta);
    
    % Align filter topology to match current/voltage sliding window
    old_p = buffer_p(idx);
    old_q = buffer_q(idx);
    
    buffer_p(idx) = p;
    buffer_q(idx) = q;
    
    sum_p = sum_p + p - old_p;
    sum_q = sum_q + q - old_q;
    
    idx = idx + 1;
    if idx > window
        idx = 1;
    end
    
    p_avg = sum_p / window;
    q_avg = sum_q / window;
    
    p_osc = p - p_avg;
    q_osc = q - q_avg;
end

== matlab function Inverter_pq_comp_sat_sim/MATLAB Function8 ==
  data: i_alpha input; p_avg output; i_beta input; v_alpha input; v_beta input; p_osc output; q_avg output; q_osc output
function [p_avg, p_osc, q_avg, q_osc] = pqCalc(i_alpha, i_beta, v_alpha, v_beta)
    % Initial logic and parameters are validated. 
    % Standard processing applied for spatial vector alignment.

    persistent buffer_p buffer_q sum_p sum_q idx
    window = 200; % Must match your 12000Hz/60Hz window size exactly
    
    if isempty(buffer_p)
        buffer_p = zeros(window, 1, "single");
        buffer_q = zeros(window, 1, "single");
        sum_p = single(0.0);
        sum_q = single(0.0);
        idx = 1;
    end
    
    % Final transformation: Strip scaling coefficients to match I_total_sq domain
    p = (v_alpha * i_alpha) + (v_beta * i_beta);
    q = (v_beta * i_alpha) - (v_alpha * i_beta);
    
    % Align filter topology to match current/voltage sliding window
    old_p = buffer_p(idx);
    old_q = buffer_q(idx);
    
    buffer_p(idx) = p;
    buffer_q(idx) = q;
    
    sum_p = sum_p + p - old_p;
    sum_q = sum_q + q - old_q;
    
    idx = idx + 1;
    if idx > window
        idx = 1;
    end
    
    p_avg = sum_p / window;
    q_avg = sum_q / window;
    
    p_osc = p - p_avg;
    q_osc = q - q_avg;
end

== matlab function Inverter_pq_comp_sat_sim/MATLAB Function9 ==
  data: lambda_Q output; lambda_PF output; i_alpha input; THDi output; i_beta input; v_alpha input; v_beta input; p_avg input; q_avg input; S_fund output
function [lambda_Q, lambda_PF, THDi, S_fund] = FOMCalc(i_alpha, i_beta, v_alpha, v_beta, p_avg, q_avg)
    % #codegen
    window = 200;
    epsilon = 1e-6;
    
    persistent buffer_I_total;
    persistent buffer_V_total;
    persistent idx;
    persistent sum_I_total;
    persistent sum_V_total;
    
    % Inicialização dos buffers na primeira amostragem
    if isempty(idx)
        buffer_I_total = zeros(window, 1, "single");
        buffer_V_total = zeros(window, 1, "single");
        idx = 1;
        sum_I_total = single(0.0);
        sum_V_total = single(0.0);
    end

    % 1. Cálculo do Fator de Deslocamento Fundamental (DPF)
    S_fund = sqrt(p_avg^2 + q_avg^2);
    if S_fund < epsilon
        lambda_Q = single(1.0);
    else
        lambda_Q = abs(p_avg) / S_fund;
    end
    
    % 2. Magnitudes Instantâneas ao Quadrado
    I_total_inst_sq = i_alpha^2 + i_beta^2;
    V_total_inst_sq = v_alpha^2 + v_beta^2;
    
    % 3. Média Móvel O(1) para os valores RMS no ciclo (Tensão e Corrente)
    old_I = buffer_I_total(idx);
    old_V = buffer_V_total(idx);
    
    buffer_I_total(idx) = I_total_inst_sq;
    buffer_V_total(idx) = V_total_inst_sq;
    
    sum_I_total = sum_I_total + I_total_inst_sq - old_I;
    sum_V_total = sum_V_total + V_total_inst_sq - old_V;
    
    idx = idx + 1;

    if idx > window
        idx = 1; 
    end
    
    I_total_sq = max(sum_I_total / window, single(0.0));
    V_total_sq = max(sum_V_total / window, single(0.0));
    
    % 4. Cálculo do Fator de Potência Total (lambda_PF)
    S_total = sqrt(V_total_sq * I_total_sq);
    
    if S_total < epsilon
        lambda_PF = single(1.0);
    else
        lambda_PF = abs(p_avg) / S_total;
    end
    
    % Saturação de segurança contra erros numéricos de arredondamento
    % lambda_PF = min(max(lambda_PF, -1.0), 1.0);
    
    % 5. Magnitude ao quadrado da Corrente Fundamental (direto da teoria p-q)
    I_fund_sq = (p_avg^2 + q_avg^2) / V_total_sq;
    
    % 6. Cálculo do THD
    diff_sq = I_total_sq - I_fund_sq;
    if diff_sq < 0
        diff_sq = single(0.0); % Proteção para pequenos erros de arredondamento
    end
    
    if I_fund_sq < epsilon
        THDi = single(0.0);
    else
        THDi = sqrt(diff_sq) / sqrt(I_fund_sq);
    end
end

== matlab function Inverter_pq_comp_sat_sim/MATLAB Function ==
  data: v_unf input; v_f output; bD input; bQ input; a1 input; a2 input; enable input
function v_f  = SOGI(v_unf, bD, bQ, a1, a2, enable)

persistent u1 u2
persistent vf1 vf2
persistent vq1 vq2

if isempty(u1)
    u1  = single(0);
    u2  = single(0);

    vf1 = single(0);
    vf2 = single(0);

    vq1 = single(0);
    vq2 = single(0);
end

if enable == 0
    u1  = single(0);
    u2  = single(0);

    vf1 = single(0);
    vf2 = single(0);

    vq1 = single(0);
    vq2 = single(0);

    v_f = single(0);
    v_q = single(0);
    return;
end

u   = single(v_unf);
bd  = single(bD);
bq  = single(bQ);
aa1 = single(a1);
aa2 = single(a2);

% In-phase band-pass output
v_f = bd*(u - u2) ...
    - aa1*vf1 ...
    - aa2*vf2;

% Quadrature output
v_q = bq*(u + single(2)*u1 + u2) ...
    - aa1*vq1 ...
    - aa2*vq2;

% Update histories AFTER calculating both outputs
u2 = u1;
u1 = u;

vf2 = vf1;
vf1 = v_f;

vq2 = vq1;
vq1 = v_q;

end

== matlab function Inverter_pq_comp_sat_sim/MATLAB Function4 ==
  data: v_unf input; v_f output; bD input; bQ input; a1 input; a2 input; enable input
function v_f  = SOGI(v_unf, bD, bQ, a1, a2, enable)

persistent u1 u2
persistent vf1 vf2
persistent vq1 vq2

if isempty(u1)
    u1  = single(0);
    u2  = single(0);

    vf1 = single(0);
    vf2 = single(0);

    vq1 = single(0);
    vq2 = single(0);
end

if enable == 0
    u1  = single(0);
    u2  = single(0);

    vf1 = single(0);
    vf2 = single(0);

    vq1 = single(0);
    vq2 = single(0);

    v_f = single(0);
    v_q = single(0);
    return;
end

u   = single(v_unf);
bd  = single(bD);
bq  = single(bQ);
aa1 = single(a1);
aa2 = single(a2);

% In-phase band-pass output
v_f = bd*(u - u2) ...
    - aa1*vf1 ...
    - aa2*vf2;

% Quadrature output
v_q = bq*(u + single(2)*u1 + u2) ...
    - aa1*vq1 ...
    - aa2*vq2;

% Update histories AFTER calculating both outputs
u2 = u1;
u1 = u;

vf2 = vf1;
vf1 = v_f;

vq2 = vq1;
vq1 = v_q;

end

== matlab function Inverter_pq_comp_sat_sim/MATLAB Function2 ==
  data: a input; alpha output; b input; c input; beta output
function [alpha, beta] = alpha_beta(a, b, c)

alpha = sqrt(2/3)*(a - b/2 - c/2);
beta  = sqrt(2/3)*(sqrt(3)*b/2 - sqrt(3)*c/2);

== matlab function Inverter_pq_comp_sat_sim/RMS_fcn ==
  data: RMSin input; yout output
function yout = fcn(RMSin)

win = 200;

persistent sampleRMS
    if isempty(sampleRMS)
        sampleRMS = single(0.0);
    end
    if sampleRMS>=win
        sampleRMS = single(0.0);
    end

persistent RMSout
if isempty(RMSout)
    RMSout = single(0.0);
end    
persistent sumRMS
if isempty(sumRMS)
    sumRMS = single(0.0);
end
persistent RMSinArray
     if isempty(RMSinArray)
         RMSinArray = zeros(1,win);
     end

sampleRMS = sampleRMS + 1;      

%RMS of Input Signal
sumRMS = sumRMS + RMSin*RMSin - RMSinArray(1,sampleRMS);
RMSinArray(1,sampleRMS) = RMSin*RMSin;
if sumRMS>=0.0
    RMSout = sqrt(sumRMS/win);
end

%RMSout = RMSout_temp;

yout = RMSout;
